simulink model "cstr_cascade"  (R2017a)
settings: Solver=ode23s  StartTime=0.0  StopTime=1199  FixedStep=0.01  RelTol=1e-10
libraries: simulink x18, commchan3 x10
settings Model: Creator=s262314  LastModifiedBy=s262314
settings DataIOCC: SaveFormat=Array  OutputOption=SpecifiedOutputTimes  OutputTimes=[0:1199]

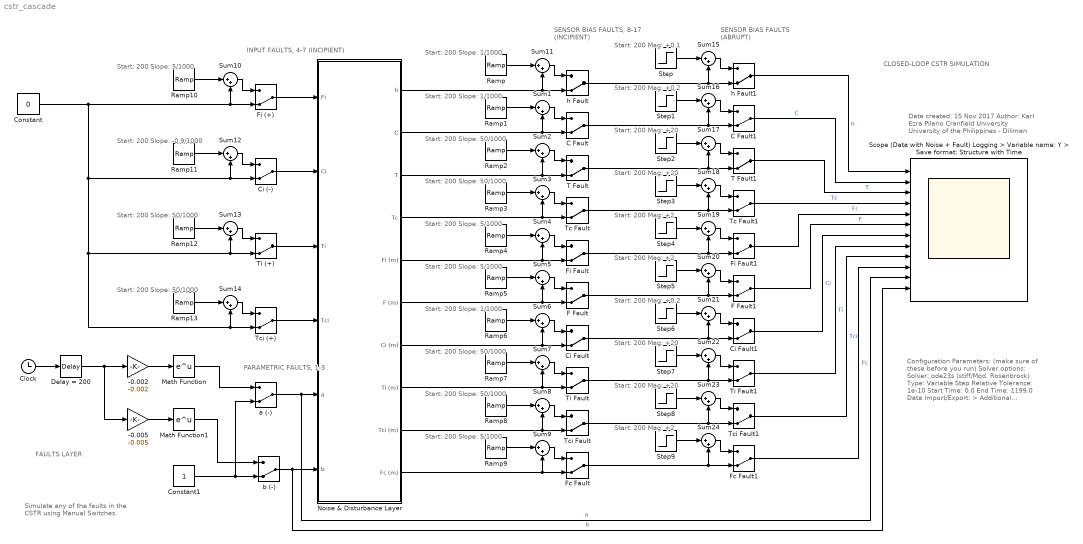
== system cstr_cascade ==
  note: Simulate any of the faults in the
      | CSTR using Manual Switches.
  note: CLOSED-LOOP
      | CSTR SIMULATION
  note: Configuration Parameters:
      | (make sure of these before you run)
      |
      | Solver options:
      | Solver: ode23s (stiff/Mod. Rosenbrock)
      | Type: Variable Step
      | Relative Tolerance: 1e-10
      | Start Time: 0.0
      | End Time: 1199.0
      |
      | Data Import/Export:
      | > Additional Parameters
      | Decimation: 1
      | > Output options:
      | Produce specified output only
      | Output times: [0:1199]
  note: Start: 200
      | Mag: +0.1
  note: Date created: 15 Nov 2017
      | Author: Karl Ezra Pilario
      | Cranfield University
      | University of the Philippines - Diliman
  note: FAULTS
      | LAYER
  note: PARAMETRIC
      | FAULTS, 1-3
  note: SENSOR BIAS
      | FAULTS, 8-17
      | (INCIPIENT)
  note: Start: 200
      | Slope: 1/1000
  note: Start: 200
      | Slope: 1/1000
  note: Start: 200
      | Slope: 50/1000
  note: Start: 200
      | Slope: 50/1000
  note: Start: 200
      | Slope: 5/1000
  note: Start: 200
      | Slope: 5/1000
  note: Start: 200
      | Slope: 1/1000
  note: Start: 200
      | Slope: 50/1000
  note: Start: 200
      | Slope: 50/1000
  note: Start: 200
      | Slope: 5/1000
  note: Start: 200
      | Slope: 5/1000
  note: INPUT
      | FAULTS, 4-7
      | (INCIPIENT)
  note: Start: 200
      | Slope: -0.9/1000
  note: Start: 200
      | Slope: 50/1000
  note: Start: 200
      | Slope: 50/1000
  note: SENSOR BIAS
      | FAULTS
      | (ABRUPT)
  note: Start: 200
      | Mag: +0.2
  note: Start: 200
      | Mag: +20
  note: Start: 200
      | Mag: +20
  note: Start: 200
      | Mag: +2
  note: Start: 200
      | Mag: +2
  note: Start: 200
      | Mag: +0.2
  note: Start: 200
      | Mag: +20
  note: Start: 200
      | Mag: +20
  note: Start: 200
      | Mag: +2
  "-0.002 " : Gain  Gain=-0.002
  -0.005 : Gain  Gain=-0.005
  C Fault : ManualSwitch  CurrentSetting=0
  C Fault1 : ManualSwitch  CurrentSetting=0
  Ci (-) : ManualSwitch  CurrentSetting=0
  Ci Fault : ManualSwitch  CurrentSetting=0
  Ci Fault1 : ManualSwitch  CurrentSetting=0
  Clock : Clock
  Constant : Constant  Value=0
  Constant1 : Constant
  Delay = 200 : TransportDelay  DelayTime=200
  F Fault : ManualSwitch  CurrentSetting=0
  F Fault1 : ManualSwitch  CurrentSetting=0
  Fc Fault : ManualSwitch  CurrentSetting=0
  Fc Fault1 : ManualSwitch  CurrentSetting=0
  Fi (+) : ManualSwitch  CurrentSetting=0
  Fi Fault : ManualSwitch  CurrentSetting=0
  Fi Fault1 : ManualSwitch  CurrentSetting=0
  Math Function : Math  SaturateOnIntegerOverflow=on
  Math Function1 : Math  SaturateOnIntegerOverflow=on
  Noise & Disturbance Layer : Subsystem
  Ramp : simulink/Sources/Ramp  slope=1/(1200-200)  start=200  X0=0
  Ramp1 : simulink/Sources/Ramp  slope=1/(1200-200)  start=200  X0=0
  Ramp{4..5,9..10} (4 alike) : simulink/Sources/Ramp  slope=5/(1200-200)  start=200  X0=0
  Ramp11 : simulink/Sources/Ramp  slope=-0.9/(1200-200)  start=200  X0=0
  Ramp{2..3,7..8,12..13} (6 alike) : simulink/Sources/Ramp  slope=50/(1200-200)  start=200  X0=0
  Ramp6 : simulink/Sources/Ramp  slope=1/(1200-200)  start=200  X0=0
  "Scope (Data with Noise + Fault) Logging > Variable name: Y > Save format: Structure with Time " : Scope  NumInputPorts=12
  Step : Step  Time=200  After=0.1  SampleTime=0
  Step1 : Step  Time=200  After=0.2  SampleTime=0
  Step{2..3,7..8} (4 alike) : Step  Time=200  After=20  SampleTime=0
  Step4 : Step  Time=200  After=2  SampleTime=0
  Step5 : Step  Time=200  After=2  SampleTime=0
  Step6 : Step  Time=200  After=0.2  SampleTime=0
  Step9 : Step  Time=200  After=2  SampleTime=0
  Sum{1..24} (24 alike) : Sum  Inputs=|++
  T Fault : ManualSwitch  CurrentSetting=0
  T Fault1 : ManualSwitch  CurrentSetting=0
  Tc Fault : ManualSwitch  CurrentSetting=0
  Tc Fault1 : ManualSwitch  CurrentSetting=0
  Tci (+) : ManualSwitch  CurrentSetting=0
  Tci Fault : ManualSwitch  CurrentSetting=0
  Tci Fault1 : ManualSwitch  CurrentSetting=0
  Ti (+) : ManualSwitch  CurrentSetting=0
  Ti Fault : ManualSwitch  CurrentSetting=0
  Ti Fault1 : ManualSwitch  CurrentSetting=0
  a (-) : ManualSwitch  CurrentSetting=0
  b (-) : ManualSwitch  CurrentSetting=0
  h Fault : ManualSwitch  CurrentSetting=0
  h Fault1 : ManualSwitch  CurrentSetting=0
  wires:
  "-0.002 "/1 -> Math Function/1
  Noise & Disturbance Layer/1(h) -> h Fault/2, Sum11/2
  Sum11/1 -> h Fault/1
  Ramp/1 -> Sum11/1
  Noise & Disturbance Layer/2(C) -> C Fault/2, Sum1/2
  Ramp1/1 -> Sum1/1
  Sum1/1 -> C Fault/1
  Noise & Disturbance Layer/3(T) -> T Fault/2, Sum2/2
  Sum2/1 -> T Fault/1
  Ramp2/1 -> Sum2/1
  Noise & Disturbance Layer/4(Tc) -> Tc Fault/2, Sum3/2
  Sum3/1 -> Tc Fault/1
  Ramp3/1 -> Sum3/1
  Sum4/1 -> Fi Fault/1
  Noise & Disturbance Layer/5(Fi (m)) -> Fi Fault/2, Sum4/2
  Ramp4/1 -> Sum4/1
  Sum5/1 -> F Fault/1
  Ramp5/1 -> Sum5/1
  Noise & Disturbance Layer/6(F (m)) -> Sum5/2, F Fault/2
  Noise & Disturbance Layer/7(Ci (m)) -> Sum6/2, Ci Fault/2
  Ramp6/1 -> Sum6/1
  Sum6/1 -> Ci Fault/1
  Ramp7/1 -> Sum7/1
  Sum7/1 -> Ti Fault/1
  Noise & Disturbance Layer/8(Ti (m)) -> Sum7/2, Ti Fault/2
  Noise & Disturbance Layer/9(Tci (m)) -> Sum8/2, Tci Fault/2
  Sum8/1 -> Tci Fault/1
  Ramp8/1 -> Sum8/1
  Noise & Disturbance Layer/10(Fc (m)) -> Sum9/2, Fc Fault/2
  Ramp9/1 -> Sum9/1
  Sum9/1 -> Fc Fault/1
  Ramp10/1 -> Sum10/1
  Sum10/1 -> Fi (+)/1
  Fi (+)/1 -> Noise & Disturbance Layer/1(Fi)
  Ramp11/1 -> Sum12/1
  Sum12/1 -> Ci (-)/1
  Ci (-)/1 -> Noise & Disturbance Layer/2(Ci)
  Sum13/1 -> Ti (+)/1
  Ramp12/1 -> Sum13/1
  Ti (+)/1 -> Noise & Disturbance Layer/3(Ti)
  Constant/1 -> Tci (+)/2, Sum14/2, Ti (+)/2, Sum13/2, Ci (-)/2, Sum12/2, Fi (+)/2, Sum10/2
  Ramp13/1 -> Sum14/1
  Sum14/1 -> Tci (+)/1
  Tci (+)/1 -> Noise & Disturbance Layer/4(Tci)
  Delay = 200/1 -> -0.005/1, "-0.002 "/1
  -0.005/1 -> Math Function1/1
  Clock/1 -> Delay = 200/1
  a (-)/1 -> Noise & Disturbance Layer/5(a), "Scope (Data with Noise + Fault) Logging > Variable name: Y > Save format: Structure with Time "/11  "a"
  b (-)/1 -> "Scope (Data with Noise + Fault) Logging > Variable name: Y > Save format: Structure with Time "/12, Noise & Disturbance Layer/6(b)  "b"
  Math Function/1 -> a (-)/1
  Math Function1/1 -> b (-)/1
  Constant1/1 -> b (-)/2, a (-)/2
  Step/1 -> Sum15/1
  Sum15/1 -> h Fault1/1
  h Fault/1 -> Sum15/2, h Fault1/2
  h Fault1/1 -> "Scope (Data with Noise + Fault) Logging > Variable name: Y > Save format: Structure with Time "/1  "h"
  Sum16/1 -> C Fault1/1
  C Fault/1 -> Sum16/2, C Fault1/2
  Step1/1 -> Sum16/1
  C Fault1/1 -> "Scope (Data with Noise + Fault) Logging > Variable name: Y > Save format: Structure with Time "/2  "C"
  Sum17/1 -> T Fault1/1
  Step2/1 -> Sum17/1
  T Fault/1 -> Sum17/2, T Fault1/2
  T Fault1/1 -> "Scope (Data with Noise + Fault) Logging > Variable name: Y > Save format: Structure with Time "/3  "T"
  Sum18/1 -> Tc Fault1/1
  Tc Fault/1 -> Sum18/2, Tc Fault1/2
  Step3/1 -> Sum18/1
  Tc Fault1/1 -> "Scope (Data with Noise + Fault) Logging > Variable name: Y > Save format: Structure with Time "/4  "Tc"
  Sum19/1 -> Fi Fault1/1
  Step4/1 -> Sum19/1
  Fi Fault/1 -> Sum19/2, Fi Fault1/2
  Fi Fault1/1 -> "Scope (Data with Noise + Fault) Logging > Variable name: Y > Save format: Structure with Time "/5  "Fi"
  F Fault/1 -> Sum20/2, F Fault1/2
  Sum20/1 -> F Fault1/1
  Step5/1 -> Sum20/1
  F Fault1/1 -> "Scope (Data with Noise + Fault) Logging > Variable name: Y > Save format: Structure with Time "/6  "F"
  Step6/1 -> Sum21/1
  Sum21/1 -> Ci Fault1/1
  Ci Fault/1 -> Sum21/2, Ci Fault1/2
  Ci Fault1/1 -> "Scope (Data with Noise + Fault) Logging > Variable name: Y > Save format: Structure with Time "/7  "Ci"
  Step7/1 -> Sum22/1
  Sum22/1 -> Ti Fault1/1
  Ti Fault/1 -> Sum22/2, Ti Fault1/2
  Ti Fault1/1 -> "Scope (Data with Noise + Fault) Logging > Variable name: Y > Save format: Structure with Time "/8  "Ti"
  Step8/1 -> Sum23/1
  Tci Fault/1 -> Sum23/2, Tci Fault1/2
  Sum23/1 -> Tci Fault1/1
  Tci Fault1/1 -> "Scope (Data with Noise + Fault) Logging > Variable name: Y > Save format: Structure with Time "/9  "Tci"
  Step9/1 -> Sum24/1
  Fc Fault/1 -> Sum24/2, Fc Fault1/2
  Sum24/1 -> Fc Fault1/1
  Fc Fault1/1 -> "Scope (Data with Noise + Fault) Logging > Variable name: Y > Save format: Structure with Time "/10  "Fc"

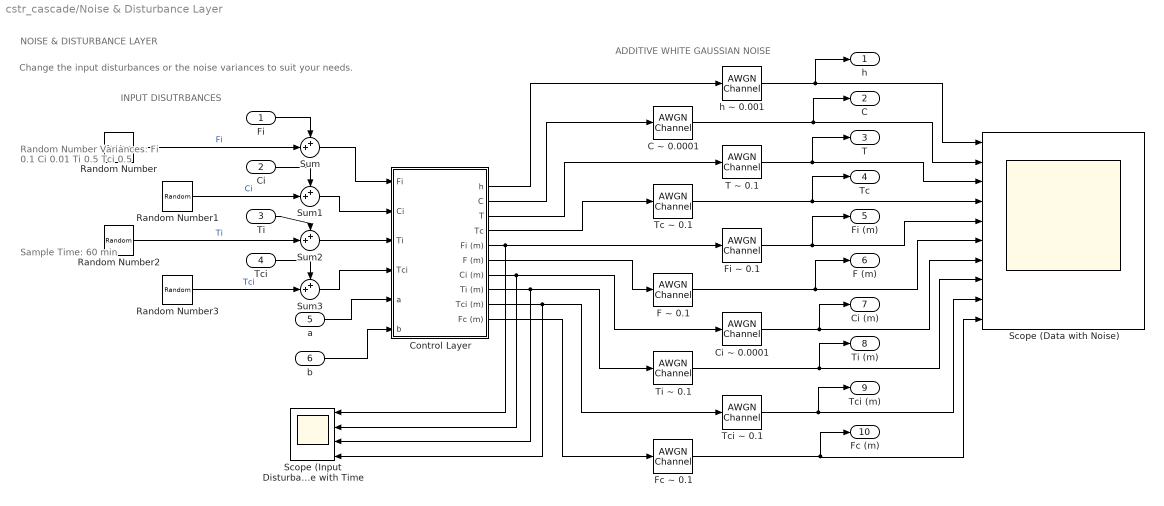
== system cstr_cascade/Noise & Disturbance Layer ==
  note: Change the input disturbances or the noise variances to suit your needs.
  note: ADDITIVE WHITE GAUSSIAN NOISE
  note: INPUT
      | DISUTRBANCES
  note: Sample Time:
      | 60 min
  note: Random
      | Number
      | Variances:
      | Fi   0.1
      | Ci   0.01
      | Ti   0.5
      | Tci  0.5
  note: NOISE & DISTURBANCE LAYER
  Fi : Inport
  Ci : Inport  Port=2
  Ti : Inport  Port=3
  Tci : Inport  Port=4
  a : Inport  Port=5
  b : Inport  Port=6
  " Tci ~ 0.1" : commchan3/AWGN Channel  InputProcessing=Columns as channels (frame based)  seed=randi(100000)  noiseMode=Variance from mask  EbNodB=100  EsNodB=10  SNRdB=10  bitsPerSym=1  Ps=1  Tsym=1  variance=0.1
  " Ti ~ 0.1" : commchan3/AWGN Channel  InputProcessing=Columns as channels (frame based)  seed=randi(100000)  noiseMode=Variance from mask  EbNodB=100  EsNodB=10  SNRdB=10  bitsPerSym=1  Ps=1  Tsym=1  variance=0.1
  C ~ 0.0001 : commchan3/AWGN Channel  InputProcessing=Columns as channels (frame based)  seed=randi(100000)  noiseMode=Variance from mask  EbNodB=100  EsNodB=10  SNRdB=10  bitsPerSym=1  Ps=1  Tsym=1  variance=0.0001
  "Ci ~ 0.0001 " : commchan3/AWGN Channel  InputProcessing=Columns as channels (frame based)  seed=randi(100000)  noiseMode=Variance from mask  EbNodB=100  EsNodB=10  SNRdB=10  bitsPerSym=1  Ps=1  Tsym=1  variance=0.0001
  Control Layer : Subsystem
  F ~ 0.1 : commchan3/AWGN Channel  InputProcessing=Columns as channels (frame based)  seed=randi(100000)  noiseMode=Variance from mask  EbNodB=100  EsNodB=10  SNRdB=10  bitsPerSym=1  Ps=1  Tsym=1  variance=0.1
  Fc ~ 0.1 : commchan3/AWGN Channel  InputProcessing=Columns as channels (frame based)  seed=randi(100000)  noiseMode=Variance from mask  EbNodB=100  EsNodB=10  SNRdB=10  bitsPerSym=1  Ps=1  Tsym=1  variance=0.1
  Fi ~ 0.1 : commchan3/AWGN Channel  InputProcessing=Columns as channels (frame based)  seed=randi(100000)  noiseMode=Variance from mask  EbNodB=100  EsNodB=10  SNRdB=10  bitsPerSym=1  Ps=1  Tsym=1  variance=0.1
  Random Number : RandomNumber  Variance=0.1  Seed=randi(100000)  SampleTime=60
  Random Number1 : RandomNumber  Variance=0.01  Seed=randi(100000)  SampleTime=60
  Random Number2 : RandomNumber  Variance=0.5  Seed=randi(100000)  SampleTime=60
  Random Number3 : RandomNumber  Variance=0.5  Seed=randi(100000)  SampleTime=60
  Scope (Data with Noise) : Scope  NumInputPorts=10
  "Scope (Input Disturbances without Noise) Logging > Variable name: U > Save format: Structure with Time " : Scope  NumInputPorts=4
  Sum{,1..3} (4 alike) : Sum  Inputs=++|
  T ~ 0.1 : commchan3/AWGN Channel  InputProcessing=Columns as channels (frame based)  seed=randi(100000)  noiseMode=Variance from mask  EbNodB=100  EsNodB=10  SNRdB=10  bitsPerSym=1  Ps=1  Tsym=1  variance=0.1
  "Tc ~ 0.1 " : commchan3/AWGN Channel  InputProcessing=Columns as channels (frame based)  seed=randi(100000)  noiseMode=Variance from mask  EbNodB=100  EsNodB=10  SNRdB=10  bitsPerSym=1  Ps=1  Tsym=1  variance=0.1
  h ~ 0.001 : commchan3/AWGN Channel  InputProcessing=Columns as channels (frame based)  seed=randi(100000)  noiseMode=Variance from mask  EbNodB=100  EsNodB=10  SNRdB=10  bitsPerSym=1  Ps=1  Tsym=1  variance=0.001
  h : Outport
  C : Outport  Port=2
  T : Outport  Port=3
  Tc : Outport  Port=4
  Fi (m) : Outport  Port=5
  F (m) : Outport  Port=6
  Ci (m) : Outport  Port=7
  Ti (m) : Outport  Port=8
  Tci (m) : Outport  Port=9
  Fc (m) : Outport  Port=10
  wires:
  " Ti ~ 0.1"/1 -> Ti (m)/1, Scope (Data with Noise)/8
  C ~ 0.0001/1 -> C/1, Scope (Data with Noise)/2
  Fi ~ 0.1/1 -> Fi (m)/1, Scope (Data with Noise)/5
  Control Layer/9(Tci (m)) -> "Scope (Input Disturbances without Noise) Logging > Variable name: U > Save format: Structure with Time "/4, " Tci ~ 0.1"/1
  Control Layer/10(Fc (m)) -> Fc ~ 0.1/1
  Control Layer/4(Tc) -> "Tc ~ 0.1 "/1
  Control Layer/3(T) -> T ~ 0.1/1
  Control Layer/1(h) -> h ~ 0.001/1
  Control Layer/5(Fi (m)) -> "Scope (Input Disturbances without Noise) Logging > Variable name: U > Save format: Structure with Time "/1, Fi ~ 0.1/1
  a/1 -> Control Layer/5(a)
  Control Layer/7(Ci (m)) -> "Scope (Input Disturbances without Noise) Logging > Variable name: U > Save format: Structure with Time "/2, "Ci ~ 0.0001 "/1
  Control Layer/8(Ti (m)) -> "Scope (Input Disturbances without Noise) Logging > Variable name: U > Save format: Structure with Time "/3, " Ti ~ 0.1"/1
  b/1 -> Control Layer/6(b)
  Control Layer/2(C) -> C ~ 0.0001/1
  Control Layer/6(F (m)) -> F ~ 0.1/1
  F ~ 0.1/1 -> F (m)/1, Scope (Data with Noise)/6
  "Tc ~ 0.1 "/1 -> Tc/1, Scope (Data with Noise)/4
  T ~ 0.1/1 -> T/1, Scope (Data with Noise)/3
  Fc ~ 0.1/1 -> Fc (m)/1, Scope (Data with Noise)/10
  "Ci ~ 0.0001 "/1 -> Ci (m)/1, Scope (Data with Noise)/7
  " Tci ~ 0.1"/1 -> Tci (m)/1, Scope (Data with Noise)/9
  h ~ 0.001/1 -> h/1, Scope (Data with Noise)/1
  Fi/1 -> Sum/1
  Sum/1 -> Control Layer/1(Fi)
  Random Number/1 -> Sum/2  "Fi"
  Sum1/1 -> Control Layer/2(Ci)
  Random Number1/1 -> Sum1/2  "Ci"
  Ci/1 -> Sum1/1
  Sum2/1 -> Control Layer/3(Ti)
  Random Number2/1 -> Sum2/2  "Ti"
  Ti/1 -> Sum2/1
  Random Number3/1 -> Sum3/2  "Tci"
  Tci/1 -> Sum3/1
  Sum3/1 -> Control Layer/4(Tci)

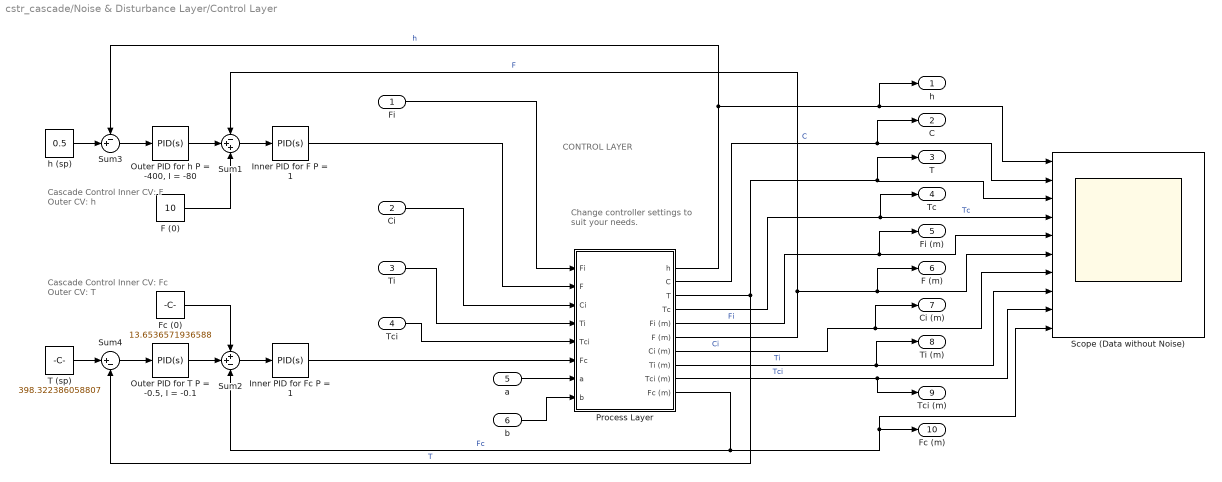
== system cstr_cascade/Noise & Disturbance Layer/Control Layer ==
  note: Change controller settings
      | to suit your needs.
  note: Cascade Control
      | Inner CV: F
      | Outer CV: h
  note: Cascade Control
      | Inner CV: Fc
      | Outer CV: T
  note: CONTROL
      | LAYER
  Fi : Inport
  Ci : Inport  Port=2
  Ti : Inport  Port=3
  Tci : Inport  Port=4
  a : Inport  Port=5
  b : Inport  Port=6
  F (0) : Constant  Value=10
  Fc (0) : Constant  Value=13.6536571936588
  Inner PID for F P = 1 : simulink/Continuous/PID Controller  Controller=PID  TimeDomain=Continuous-time  SampleTime=-1  IntegratorMethod=Forward Euler  FilterMethod=Forward Euler  Form=Parallel  UseFilter=on  ControllerParametersSource=internal  P=1  I=0  D=0  N=100  InitialConditionSource=internal  InitialConditionForIntegrator=0  InitialConditionForFilter=0  ExternalReset=none  LimitOutput=off  UpperSaturationLimit=inf  LowerSaturationLimit=-inf  LinearizeAsGain=on  AntiWindupMode=none  Kb=1  TrackingMode=off  Kt=1  PParamMin=[]  PParamMax=[]  IParamMin=[]  IParamMax=[]  DParamMin=[]  DParamMax=[]  NParamMin=[]  NParamMax=[]  KbParamMin=[]  KbParamMax=[]  KtParamMin=[]  KtParamMax=[]  POutMin=[]  POutMax=[]  IOutMin=[]  IOutMax=[]  DOutMin=[]  DOutMax=[]  NOutMin=[]  NOutMax=[]  KbOutMin=[]  KbOutMax=[]  KtOutMin=[]  KtOutMax=[]  IntegratorOutMin=[]  IntegratorOutMax=[]  FilterOutMin=[]  FilterOutMax=[]  SumOutMin=[]  SumOutMax=[]  SumI1OutMin=[]  SumI1OutMax=[]  SumI2OutMin=[]  SumI2OutMax=[]  SumI3OutMin=[]  SumI3OutMax=[]  SumDOutMin=[]  SumDOutMax=[]  SaturationOutMin=[]  SaturationOutMax=[]  IntegratorContinuousStateAttributes=''  IntegratorStateMustResolveToSignalObject=off  IntegratorRTWStateStorageClass=Auto  FilterContinuousStateAttributes=''  FilterStateMustResolveToSignalObject=off  FilterRTWStateStorageClass=Auto  DifferentiatorICPrevScaledInput=0  DifferentiatorOutMin=[]  DifferentiatorOutMax=[]  InitialConditionSetting=State (most efficient)
  Inner PID for Fc P = 1 : simulink/Continuous/PID Controller  Controller=PID  TimeDomain=Continuous-time  SampleTime=-1  IntegratorMethod=Forward Euler  FilterMethod=Forward Euler  Form=Parallel  UseFilter=on  ControllerParametersSource=internal  P=1  I=0  D=0  N=100  InitialConditionSource=internal  InitialConditionForIntegrator=0  InitialConditionForFilter=0  ExternalReset=none  LimitOutput=off  UpperSaturationLimit=inf  LowerSaturationLimit=-inf  LinearizeAsGain=on  AntiWindupMode=none  Kb=1  TrackingMode=off  Kt=1  PParamMin=[]  PParamMax=[]  IParamMin=[]  IParamMax=[]  DParamMin=[]  DParamMax=[]  NParamMin=[]  NParamMax=[]  KbParamMin=[]  KbParamMax=[]  KtParamMin=[]  KtParamMax=[]  POutMin=[]  POutMax=[]  IOutMin=[]  IOutMax=[]  DOutMin=[]  DOutMax=[]  NOutMin=[]  NOutMax=[]  KbOutMin=[]  KbOutMax=[]  KtOutMin=[]  KtOutMax=[]  IntegratorOutMin=[]  IntegratorOutMax=[]  FilterOutMin=[]  FilterOutMax=[]  SumOutMin=[]  SumOutMax=[]  SumI1OutMin=[]  SumI1OutMax=[]  SumI2OutMin=[]  SumI2OutMax=[]  SumI3OutMin=[]  SumI3OutMax=[]  SumDOutMin=[]  SumDOutMax=[]  SaturationOutMin=[]  SaturationOutMax=[]  IntegratorContinuousStateAttributes=''  IntegratorStateMustResolveToSignalObject=off  IntegratorRTWStateStorageClass=Auto  FilterContinuousStateAttributes=''  FilterStateMustResolveToSignalObject=off  FilterRTWStateStorageClass=Auto  DifferentiatorICPrevScaledInput=0  DifferentiatorOutMin=[]  DifferentiatorOutMax=[]  InitialConditionSetting=State (most efficient)
  "Outer PID for T P = -0.5, I = -0.1" : simulink/Continuous/PID Controller  Controller=PID  TimeDomain=Continuous-time  SampleTime=-1  IntegratorMethod=Forward Euler  FilterMethod=Forward Euler  Form=Parallel  UseFilter=on  ControllerParametersSource=internal  P=-0.5  I=-0.1  D=0  N=100  InitialConditionSource=internal  InitialConditionForIntegrator=0  InitialConditionForFilter=0  ExternalReset=none  LimitOutput=off  UpperSaturationLimit=inf  LowerSaturationLimit=-inf  LinearizeAsGain=on  AntiWindupMode=none  Kb=1  TrackingMode=off  Kt=1  PParamMin=[]  PParamMax=[]  IParamMin=[]  IParamMax=[]  DParamMin=[]  DParamMax=[]  NParamMin=[]  NParamMax=[]  KbParamMin=[]  KbParamMax=[]  KtParamMin=[]  KtParamMax=[]  POutMin=[]  POutMax=[]  IOutMin=[]  IOutMax=[]  DOutMin=[]  DOutMax=[]  NOutMin=[]  NOutMax=[]  KbOutMin=[]  KbOutMax=[]  KtOutMin=[]  KtOutMax=[]  IntegratorOutMin=[]  IntegratorOutMax=[]  FilterOutMin=[]  FilterOutMax=[]  SumOutMin=[]  SumOutMax=[]  SumI1OutMin=[]  SumI1OutMax=[]  SumI2OutMin=[]  SumI2OutMax=[]  SumI3OutMin=[]  SumI3OutMax=[]  SumDOutMin=[]  SumDOutMax=[]  SaturationOutMin=[]  SaturationOutMax=[]  IntegratorContinuousStateAttributes=''  IntegratorStateMustResolveToSignalObject=off  IntegratorRTWStateStorageClass=Auto  FilterContinuousStateAttributes=''  FilterStateMustResolveToSignalObject=off  FilterRTWStateStorageClass=Auto  DifferentiatorICPrevScaledInput=0  DifferentiatorOutMin=[]  DifferentiatorOutMax=[]  InitialConditionSetting=State (most efficient)
  "Outer PID for h P = -400, I = -80" : simulink/Continuous/PID Controller  Controller=PID  TimeDomain=Continuous-time  SampleTime=-1  IntegratorMethod=Forward Euler  FilterMethod=Forward Euler  Form=Parallel  UseFilter=on  ControllerParametersSource=internal  P=-400  I=-80  D=0  N=100  InitialConditionSource=internal  InitialConditionForIntegrator=0  InitialConditionForFilter=0  ExternalReset=none  LimitOutput=off  UpperSaturationLimit=inf  LowerSaturationLimit=-inf  LinearizeAsGain=on  AntiWindupMode=none  Kb=1  TrackingMode=off  Kt=1  PParamMin=[]  PParamMax=[]  IParamMin=[]  IParamMax=[]  DParamMin=[]  DParamMax=[]  NParamMin=[]  NParamMax=[]  KbParamMin=[]  KbParamMax=[]  KtParamMin=[]  KtParamMax=[]  POutMin=[]  POutMax=[]  IOutMin=[]  IOutMax=[]  DOutMin=[]  DOutMax=[]  NOutMin=[]  NOutMax=[]  KbOutMin=[]  KbOutMax=[]  KtOutMin=[]  KtOutMax=[]  IntegratorOutMin=[]  IntegratorOutMax=[]  FilterOutMin=[]  FilterOutMax=[]  SumOutMin=[]  SumOutMax=[]  SumI1OutMin=[]  SumI1OutMax=[]  SumI2OutMin=[]  SumI2OutMax=[]  SumI3OutMin=[]  SumI3OutMax=[]  SumDOutMin=[]  SumDOutMax=[]  SaturationOutMin=[]  SaturationOutMax=[]  IntegratorContinuousStateAttributes=''  IntegratorStateMustResolveToSignalObject=off  IntegratorRTWStateStorageClass=Auto  FilterContinuousStateAttributes=''  FilterStateMustResolveToSignalObject=off  FilterRTWStateStorageClass=Auto  DifferentiatorICPrevScaledInput=0  DifferentiatorOutMin=[]  DifferentiatorOutMax=[]  InitialConditionSetting=State (most efficient)
  Process Layer : Subsystem
  Scope (Data without Noise) : Scope  NumInputPorts=10
  Sum1 : Sum  Inputs=-++
  Sum2 : Sum  Inputs=++-
  Sum3 : Sum  Inputs=-+|
  Sum4 : Sum  Inputs=|+-
  T (sp) : Constant  Value=398.322386058807
  h (sp) : Constant  Value=0.5
  h : Outport
  C : Outport  Port=2
  T : Outport  Port=3
  Tc : Outport  Port=4
  Fi (m) : Outport  Port=5
  F (m) : Outport  Port=6
  Ci (m) : Outport  Port=7
  Ti (m) : Outport  Port=8
  Tci (m) : Outport  Port=9
  Fc (m) : Outport  Port=10
  wires:
  "Outer PID for h P = -400, I = -80"/1 -> Sum1/2
  Sum3/1 -> "Outer PID for h P = -400, I = -80"/1
  Process Layer/7(Ci (m)) -> Ci (m)/1, Scope (Data without Noise)/7  "Ci"
  Process Layer/4(Tc) -> Tc/1, Scope (Data without Noise)/4  "Tc"
  a/1 -> Process Layer/7(a)
  Ci/1 -> Process Layer/3(Ci)
  Ti/1 -> Process Layer/4(Ti)
  b/1 -> Process Layer/8(b)
  Inner PID for F P = 1/1 -> Process Layer/2(F)
  Process Layer/3(T) -> Sum4/2, T/1, Scope (Data without Noise)/3  "T"
  Process Layer/2(C) -> C/1, Scope (Data without Noise)/2  "C"
  Process Layer/9(Tci (m)) -> Tci (m)/1, Scope (Data without Noise)/9  "Tci"
  Process Layer/6(F (m)) -> F (m)/1, Scope (Data without Noise)/6, Sum1/1  "F"
  Process Layer/5(Fi (m)) -> Fi (m)/1, Scope (Data without Noise)/5  "Fi"
  Process Layer/10(Fc (m)) -> Sum2/3, Fc (m)/1, Scope (Data without Noise)/10  "Fc"
  Process Layer/8(Ti (m)) -> Ti (m)/1, Scope (Data without Noise)/8  "Ti"
  "Outer PID for T P = -0.5, I = -0.1"/1 -> Sum2/2
  Tci/1 -> Process Layer/5(Tci)
  Inner PID for Fc P = 1/1 -> Process Layer/6(Fc)
  h (sp)/1 -> Sum3/2
  T (sp)/1 -> Sum4/1
  Fi/1 -> Process Layer/1(Fi)
  Process Layer/1(h) -> Sum3/1, h/1, Scope (Data without Noise)/1  "h"
  Sum1/1 -> Inner PID for F P = 1/1
  F (0)/1 -> Sum1/3
  Fc (0)/1 -> Sum2/1
  Sum2/1 -> Inner PID for Fc P = 1/1
  Sum4/1 -> "Outer PID for T P = -0.5, I = -0.1"/1

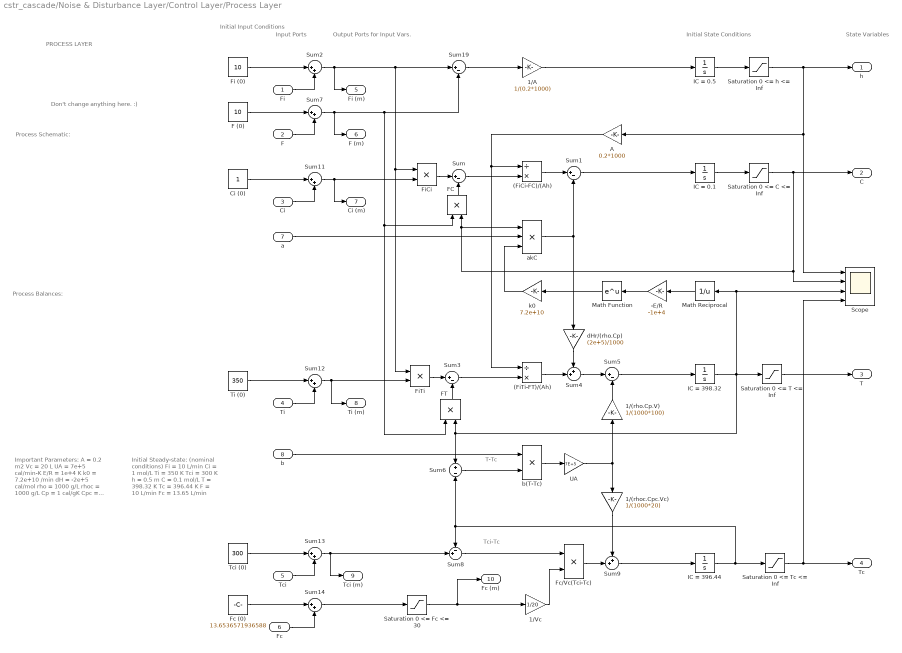
== system cstr_cascade/Noise & Disturbance Layer/Control Layer/Process Layer ==
  note: Don't change anything here. :)
  note: Process Schematic:
  note: PROCESS
      | LAYER
  note: Output Ports
      | for Input Vars.
  note: Initial State
      | Conditions
  note: State
      | Variables
  note: Input
      | Ports
  note: Initial Input
      | Conditions
  note: Initial Steady-state:
      | (nominal conditions)
      |
      | Fi = 10 L/min
      | Ci = 1 mol/L
      | Ti = 350 K
      | Tci = 300 K
      |
      | h = 0.5 m
      | C = 0.1 mol/L
      | T = 398.32 K
      | Tc = 396.44 K
      | F = 10 L/min
      | Fc = 13.65 L/min
  note: Tci-Tc
  note: T-Tc
  note: Important Parameters:
      |
      | A = 0.2 m2
      | Vc = 20 L
      | UA = 7e+5 cal/min-K
      | E/R = 1e+4 K
      | k0 = 7.2e+10 /min
      | dH = -2e+5 cal/mol
      | rho = 1000 g/L
      | rhoc = 1000 g/L
      | Cp = 1 cal/gK
      | Cpc = 1 cal/gK
      | a = 1 (catalyst activity)
      | b = 1 (heat transfer)
  note: Process Balances:
  Fi : Inport
  F : Inport  Port=2
  Ci : Inport  Port=3
  Ti : Inport  Port=4
  Tci : Inport  Port=5
  Fc : Inport  Port=6
  a : Inport  Port=7
  b : Inport  Port=8
  (FiCi-FC)/(Ah) : Product  Inputs=/*
  (FiTi-FT)/(Ah) : Product  Inputs=/*
  -E/R : Gain  Gain=-1e+4
  1/(rho.Cp.V) : Gain  Gain=1/(1000*100)
  1/(rhoc.Cpc.Vc) : Gain  Gain=1/(1000*20)
  1/A : Gain  Gain=1/(0.2*1000)
  1/Vc : Gain  Gain=1/20
  A : Gain  Gain=0.2*1000
  Ci (0) : Constant
  F (0) : Constant  Value=10
  FC : Product
  FT : Product
  Fc (0) : Constant  Value=13.6536571936588
  Fc/Vc(Tci-Tc) : Product
  Fi (0) : Constant  Value=10
  FiCi : Product
  FiTi : Product
  IC = 0.1 : Integrator  InitialCondition=0.1
  IC = 0.5 : Integrator  InitialCondition=0.5
  IC = 396.44 : Integrator  InitialCondition=396.441277288219
  IC = 398.32 : Integrator  InitialCondition=398.322386058807
  Math Function : Math  SaturateOnIntegerOverflow=on
  Math Reciprocal : Math  Operator=reciprocal  SaturateOnIntegerOverflow=on
  Saturation 0 <= C <= Inf : Saturate  UpperLimit=Inf  LowerLimit=0
  Saturation 0 <= Fc <= 30 : Saturate  UpperLimit=30  LowerLimit=0
  Saturation 0 <= T <= Inf : Saturate  UpperLimit=Inf  LowerLimit=0
  Saturation 0 <= Tc <= Inf : Saturate  UpperLimit=Inf  LowerLimit=0
  Saturation 0 <= h <= Inf : Saturate  UpperLimit=Inf  LowerLimit=0
  Scope : Scope  NumInputPorts=4
  Sum{,1,3,5,19} (5 alike) : Sum  Inputs=|+-
  Sum{2,7,11..14} (6 alike) : Sum  Inputs=|++
  Sum4 : Sum  Inputs=++|
  Sum6 : Sum  Inputs=+|-
  Sum8 : Sum  Inputs=-+|
  Sum9 : Sum  Inputs=++|
  Tci (0) : Constant  Value=300
  Ti (0) : Constant  Value=350
  UA : Gain  Gain=7E+5
  akC : Product  Inputs=3
  b(T-Tc) : Product
  dHr/(rho.Cp) : Gain  Gain=(2e+5)/1000
  k0 : Gain  Gain=7.2e+10
  h : Outport
  C : Outport  Port=2
  T : Outport  Port=3
  Tc : Outport  Port=4
  Fi (m) : Outport  Port=5
  F (m) : Outport  Port=6
  Ci (m) : Outport  Port=7
  Ti (m) : Outport  Port=8
  Tci (m) : Outport  Port=9
  Fc (m) : Outport  Port=10
  wires:
  Sum/1 -> (FiCi-FC)/(Ah)/2
  Math Function/1 -> k0/1
  Fc (0)/1 -> Sum14/1
  Saturation 0 <= Fc <= 30/1 -> Fc (m)/1, 1/Vc/1
  IC = 398.32/1 -> Saturation 0 <= T <= Inf/1, Math Reciprocal/1, Scope/3, Sum6/1, FT/2
  Sum19/1 -> 1/A/1
  Ci (0)/1 -> Sum11/1
  Math Reciprocal/1 -> -E/R/1
  1/Vc/1 -> Fc/Vc(Tci-Tc)/2
  Sum8/1 -> Fc/Vc(Tci-Tc)/1
  Sum2/1 -> Fi (m)/1, FiTi/1, FiCi/1, Sum19/1
  -E/R/1 -> Math Function/1
  IC = 0.1/1 -> Saturation 0 <= C <= Inf/1
  1/A/1 -> IC = 0.5/1
  Sum3/1 -> (FiTi-FT)/(Ah)/2
  Ci/1 -> Sum11/2
  (FiCi-FC)/(Ah)/1 -> Sum1/1
  Fc/Vc(Tci-Tc)/1 -> Sum9/2
  Sum5/1 -> IC = 398.32/1
  Sum4/1 -> Sum5/1
  Fc/1 -> Sum14/2
  FT/1 -> Sum3/2
  FC/1 -> Sum/2
  Ti/1 -> Sum12/2
  Sum9/1 -> IC = 396.44/1
  Sum1/1 -> IC = 0.1/1
  Tci (0)/1 -> Sum13/1
  FiTi/1 -> Sum3/1
  A/1 -> (FiTi-FT)/(Ah)/1, (FiCi-FC)/(Ah)/1
  Tci/1 -> Sum13/2
  IC = 396.44/1 -> Saturation 0 <= Tc <= Inf/1, Sum8/1, Sum6/2
  1/(rhoc.Cpc.Vc)/1 -> Sum9/1
  IC = 0.5/1 -> Saturation 0 <= h <= Inf/1
  k0/1 -> akC/3
  FiCi/1 -> Sum/1
  1/(rho.Cp.V)/1 -> Sum5/2
  UA/1 -> 1/(rho.Cp.V)/1, 1/(rhoc.Cpc.Vc)/1
  Sum11/1 -> FiCi/2, Ci (m)/1
  akC/1 -> Sum1/2, dHr/(rho.Cp)/1
  a/1 -> akC/2
  (FiTi-FT)/(Ah)/1 -> Sum4/2
  b(T-Tc)/1 -> UA/1
  dHr/(rho.Cp)/1 -> Sum4/1
  Ti (0)/1 -> Sum12/1
  Sum14/1 -> Saturation 0 <= Fc <= 30/1
  Fi/1 -> Sum2/2
  Fi (0)/1 -> Sum2/1
  Sum6/1 -> b(T-Tc)/2
  b/1 -> b(T-Tc)/1
  Sum12/1 -> Ti (m)/1, FiTi/2
  Sum13/1 -> Sum8/2, Tci (m)/1
  Saturation 0 <= h <= Inf/1 -> h/1, Scope/1, A/1
  Saturation 0 <= C <= Inf/1 -> C/1, Scope/2, akC/1, FC/2
  Saturation 0 <= T <= Inf/1 -> T/1
  Saturation 0 <= Tc <= Inf/1 -> Tc/1, Scope/4
  F/1 -> Sum7/2
  Sum7/1 -> F (m)/1, FC/1, FT/1, Sum19/2
  F (0)/1 -> Sum7/1
